simulink model "regbot_1mg_full"  (R2022b)
settings: Solver=ode15s  StartTime=0.0  StopTime=30  MaxStep=0.001  RelTol=1e-3  EnableMultiTasking=on
undefined symbols (not defined in the file or in its folder): alphaRT, alphaXV, BA, JA, K_PRT, K_PTV, K_PXV, Kemf, Kffwv, Kpwv, LA, mframe, mmotor, mtopextra, NG, pushDist, RA, startAngle, tau_dRT, tau_dTV, tau_dXV, tau_filter, tau_iRT, tau_iTV, tau_iXV, tau_post, tiwv, twvlp, WR, X, Y, Z
libraries: sm_lib x18, nesl_utility x9
settings Model: Creator=chr  LastModifiedBy=andre
settings SolverCC: AlgebraicLoopSolver=TrustRegion
settings DataIOCC: LimitDataPoints=on  SaveFormat=Array  ReturnWorkspaceOutputs=off
settings OptimizationCC: ExpressionDepthLimit=2147483647  LifeSpan=inf
settings DebuggingCC: UnderspecifiedInitializationDetection=Classic  MergeDetectMultiDrivingBlocksExec=none  SolverPrmCheckMsg=warning  UnconnectedInputMsg=warning  UnconnectedOutputMsg=warning  UnconnectedLineMsg=warning  StateNameClashWarn=warning  SFUnexpectedBacktrackingDiag=warning  SFNoUnconditionalDefaultTransitionDiag=warning  SFExecutionAtInitializationDiag=none  ArithmeticOperatorsInVariantConditions=warning
settings HardwareCC: ProdBitPerPointer=32  ProdBitPerSizeT=32  ProdBitPerPtrDiffT=32  ProdLargestAtomicFloat=None  ProdIntDivRoundTo=Undefined  ProdEndianess=Unspecified  ProdWordSize=32  ProdHWDeviceType=32-bit Generic
settings ModelReferenceCC: EnableRefExpFcnMdlSchedulingChecks=on  PropagateSignalLabelsOutOfModel=off
settings SFSimCC: SimUseLocalCustomCode=off  CustomCodeUndefinedFunction=UseInterfaceOnly
settings RTWCC: RTWUseLocalCustomCode=off  DLArmComputeVersion=19.05
settings CodeAppCC: StateflowObjectComments=on
settings GRTTargetCC: TargetLangStandard=C89/C90 (ANSI)
settings ConfigComp: CovMetricSettings=dw  CovSaveCumulativeToWorkspaceVar=on  CovSaveSingleToWorkspaceVar=on  CovExternalEMLEnable=off
settings SimscapeCC: SimscapeNormalizeSystem=off
settings ConfigurationSet: Description=SimMechanics 2G

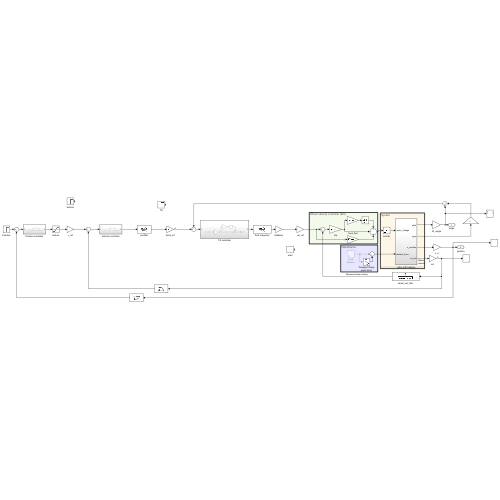
[thumbnail: Simulink's stored preview of the top-level diagram]
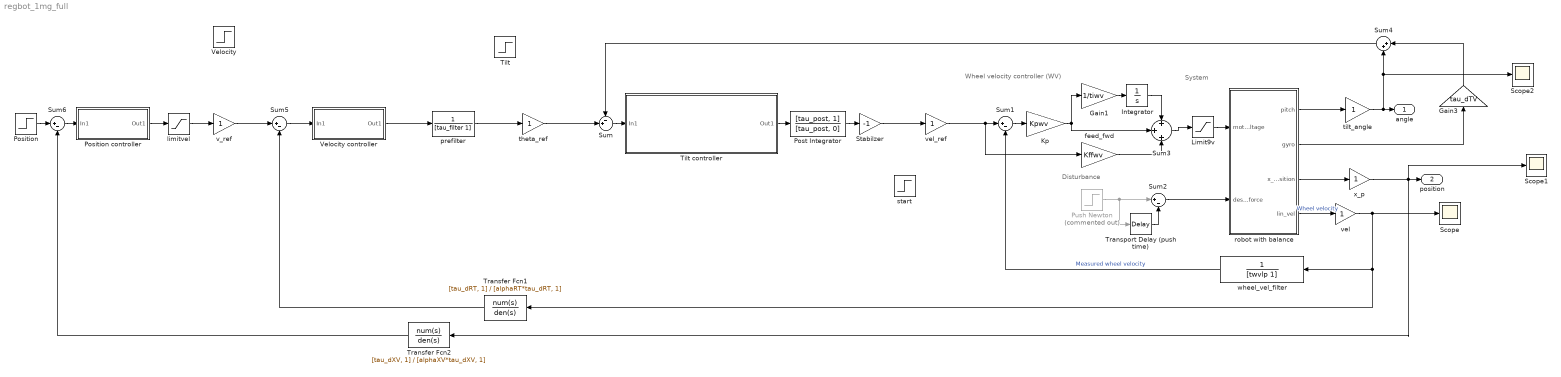
== system regbot_1mg_full ==
  note: System
  note: Disturbance
  note: Wheel velocity controller (WV)
  Gain1 : Gain  Gain=1/tiwv
  Gain3 : Gain  Gain=tau_dTV
  Integrator : Integrator  LimitOutput=on  UpperSaturationLimit=3  LowerSaturationLimit=-3
  Kp : Gain  Gain=Kpwv
  Limit9v : Saturate  UpperLimit=9  LowerLimit=-9
  Position : Step  Time=0  After=5  SampleTime=0
  Position controller : Subsystem
  Post Integrator : TransferFcn  Numerator=[tau_post, 1]  Denominator=[tau_post, 0]
  Push Newton : Step  Commented=on  After=2  SampleTime=0
  Scope : Scope
  Scope1 : Scope
  Scope2 : Scope
  Stabilzer : Gain  Gain=-1
  Sum : Sum  Inputs=-+|
  Sum{1..2,5..6} (4 alike) : Sum  Inputs=|+-
  Sum3 : Sum  Inputs=+|+|+
  Sum4 : Sum  Inputs=|++
  Tilt : Step  Time=0.2  After=3*pi/180  SampleTime=0
  Tilt controller : Subsystem
  Transfer Fcn1 : TransferFcn  Numerator=[tau_dRT, 1]  Denominator=[alphaRT*tau_dRT, 1]
  Transfer Fcn2 : TransferFcn  Numerator=[tau_dXV, 1]  Denominator=[alphaXV*tau_dXV, 1]
  Transport Delay (push time) : TransportDelay  DelayTime=0.1
  Velocity : Step  Time=0  After=0.8  SampleTime=0
  Velocity controller : Subsystem
  feed_fwd : Gain  Gain=Kffwv
  limitvel : Saturate  UpperLimit=1.2  LowerLimit=-1.2
  prefilter : TransferFcn  Denominator=[tau_filter 1]
  robot with balance : Subsystem
  start : Step  Time=0.2  After=1.1  SampleTime=0
  theta_ref : Gain
  tilt_angle : Gain
  v_ref : Gain
  vel : Gain
  vel_ref : Gain
  wheel_vel_filter : TransferFcn  Denominator=[twvlp 1]
  x_p : Gain
  angle : Outport  VectorParamsAs1DForOutWhenUnconnected=off
  position : Outport  Port=2  VectorParamsAs1DForOutWhenUnconnected=off
  wires:
  Push Newton/1 -> Transport Delay (push time)/1, Sum2/1
  Sum2/1 -> robot with balance/2(desturb_force)
  Transport Delay (push time)/1 -> Sum2/2
  Limit9v/1 -> robot with balance/1(motor_Voltage)
  Sum1/1 -> Kp/1
  Gain1/1 -> Integrator/1
  Integrator/1 -> Sum3/1
  Kp/1 -> Gain1/1, Sum3/2
  Sum3/1 -> Limit9v/1
  robot with balance/1(pitch) -> tilt_angle/1
  feed_fwd/1 -> Sum3/3
  wheel_vel_filter/1 -> Sum1/2  "Measured wheel velocity"
  vel_ref/1 -> feed_fwd/1, Sum1/1
  tilt_angle/1 -> Sum4/2, Scope2/1, angle/1
  Post Integrator/1 -> Stabilzer/1
  robot with balance/2(gyro) -> Gain3/1
  Sum4/1 -> Sum/1
  Sum/1 -> Tilt controller/1(In1)
  Gain3/1 -> Sum4/1
  Tilt controller/1(Out1) -> Post Integrator/1
  theta_ref/1 -> Sum/2
  Sum5/1 -> Velocity controller/1(In1)
  robot with balance/4(lin_vel) -> vel/1  "Wheel velocity"
  vel/1 -> Scope/1, Transfer Fcn1/1, wheel_vel_filter/1
  Velocity controller/1(Out1) -> prefilter/1
  Transfer Fcn1/1 -> Sum5/2
  robot with balance/3(x_position) -> x_p/1
  x_p/1 -> Scope1/1, position/1, Transfer Fcn2/1
  Position/1 -> Sum6/1
  Sum6/1 -> Position controller/1(In1)
  Transfer Fcn2/1 -> Sum6/2
  v_ref/1 -> Sum5/1
  Stabilzer/1 -> vel_ref/1
  prefilter/1 -> theta_ref/1
  Position controller/1(Out1) -> limitvel/1
  limitvel/1 -> v_ref/1

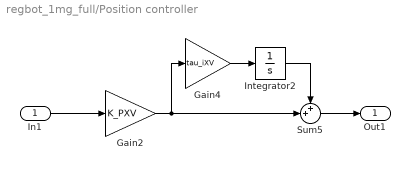
== system regbot_1mg_full/Position controller ==
  In1 : Inport
  Gain2 : Gain  Gain=K_PXV
  Gain4 : Gain  Gain=tau_iXV
  Integrator2 : Integrator  LimitOutput=on  UpperSaturationLimit=3  LowerSaturationLimit=-3
  Sum5 : Sum  Inputs=++|
  Out1 : Outport
  wires:
  Sum5/1 -> Out1/1
  In1/1 -> Gain2/1
  Gain4/1 -> Integrator2/1
  Gain2/1 -> Sum5/2, Gain4/1
  Integrator2/1 -> Sum5/1

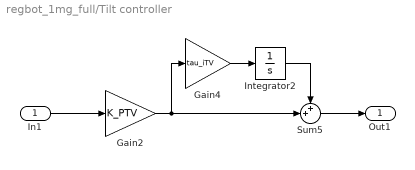
== system regbot_1mg_full/Tilt controller ==
  In1 : Inport
  Gain2 : Gain  Gain=K_PTV
  Gain4 : Gain  Gain=tau_iTV
  Integrator2 : Integrator  LimitOutput=on  UpperSaturationLimit=3  LowerSaturationLimit=-3
  Sum5 : Sum  Inputs=++|
  Out1 : Outport
  wires:
  Gain2/1 -> Gain4/1, Sum5/2
  Integrator2/1 -> Sum5/1
  Gain4/1 -> Integrator2/1
  Sum5/1 -> Out1/1
  In1/1 -> Gain2/1

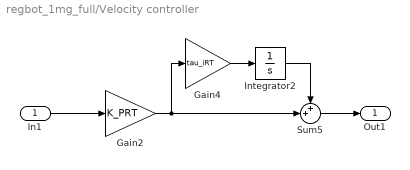
== system regbot_1mg_full/Velocity controller ==
  In1 : Inport
  Gain2 : Gain  Gain=K_PRT
  Gain4 : Gain  Gain=tau_iRT
  Integrator2 : Integrator  LimitOutput=on  UpperSaturationLimit=3  LowerSaturationLimit=-3
  Sum5 : Sum  Inputs=++|
  Out1 : Outport
  wires:
  Sum5/1 -> Out1/1
  In1/1 -> Gain2/1
  Gain4/1 -> Integrator2/1
  Gain2/1 -> Sum5/2, Gain4/1
  Integrator2/1 -> Sum5/1

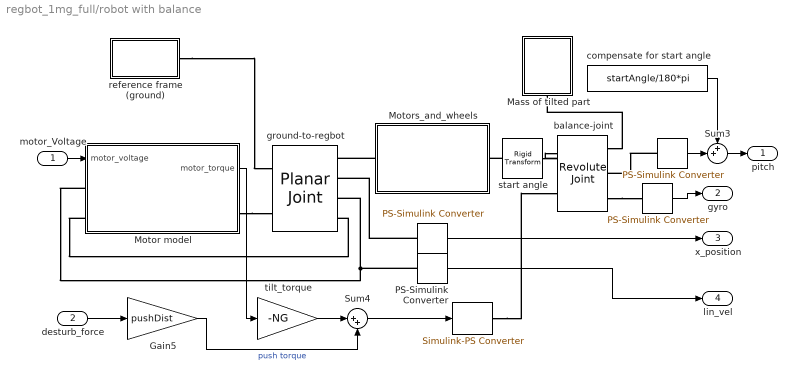
== system regbot_1mg_full/robot with balance ==
  motor_Voltage : Inport
  desturb_force : Inport  Port=2
  " " : nesl_utility/PS-Simulink Converter  PhysicalDomain=network_engine_domain  SubClassName=ps_output  LeftPortType=input  RightPortType=output  PseudoPeriodic=off  Frequencies=[]  VectorFormat=1-D array  Unit=1  AffineConversion=off
  "  " : nesl_utility/PS-Simulink Converter  PhysicalDomain=network_engine_domain  SubClassName=ps_output  LeftPortType=input  RightPortType=output  PseudoPeriodic=off  Frequencies=[]  VectorFormat=1-D array  Unit=1  AffineConversion=off
  "   " : nesl_utility/Simulink-PS Converter  PhysicalDomain=network_engine_domain  SubClassName=ps_input  LeftPortType=input  RightPortType=output  PseudoPeriodic=off  Frequencies=[]  NoiseDistribution=none  NoiseParameters=[]  Unit=1  AffineConversion=off  FilteringAndDerivatives=zero  SimscapeFilterOrder=1  InputFilterTimeConstant=.001  UdotUserProvided=[]
  "     " : nesl_utility/PS-Simulink Converter  PhysicalDomain=network_engine_domain  SubClassName=ps_output  LeftPortType=input  RightPortType=output  PseudoPeriodic=off  Frequencies=[]  VectorFormat=1-D array  Unit=1  AffineConversion=off
  Gain5 : Gain  Gain=pushDist
  Mass of tilted part : Subsystem
  Motor model : Subsystem
  Motors_and_wheels : Subsystem
  PS-Simulink Converter : nesl_utility/PS-Simulink Converter  PhysicalDomain=network_engine_domain  SubClassName=ps_output  LeftPortType=input  RightPortType=output  PseudoPeriodic=off  Frequencies=[]  VectorFormat=1-D array  Unit=1  AffineConversion=off
  Sum3 : Sum  Inputs=++|
  Sum4 : Sum  Inputs=|++
  balance-joint : sm_lib/Joints/Revolute Joint  JointMode=Normal  SenseConstraintForce=off  SenseConstraintForceX=off  SenseConstraintForceY=off  SenseConstraintForceZ=off  SenseConstraintTorque=off  SenseConstraintTorqueX=off  SenseConstraintTorqueY=off  SenseConstraintTorqueZ=off  SenseTotalForce=off  SenseTotalForceX=off  SenseTotalForceY=off  SenseTotalForceZ=off  SenseTotalTorque=off  SenseTotalTorqueX=off  SenseTotalTorqueY=off  SenseTotalTorqueZ=off  CompositeWrenchDir=FollowerOnBase  CompositeWrenchFrame=BaseFrame  EquilibriumPosition=0  EquilibriumPositionUnits=deg  SpringStiffness=0  SpringStiffnessUnits=N*m/deg  DampingCoefficient=0  DampingCoefficientUnits=N*m/(deg/s)  TorqueActuationMode=InputTorque  MotionActuationMode=ComputedMotion  SensePosition=on  SenseVelocity=on  SenseAcceleration=off  SenseTorqueForce=off  SenseLowerLimitTorqueForce=off  SenseUpperLimitTorqueForce=off  LowerLimitSpecify=off  LowerLimitBound=-90  LowerLimitBoundUnits=deg  LowerLimitStiffness=1e4  LowerLimitStiffnessUnits=N*m/deg  LowerLimitDamping=10  LowerLimitDampingUnits=N*m/(deg/s)  LowerLimitTransitionRegionWidth=0.1  LowerLimitTransitionRegionWidthUnits=deg  UpperLimitSpecify=off  UpperLimitBound=90  UpperLimitBoundUnits=deg  UpperLimitStiffness=1e4  UpperLimitStiffnessUnits=N*m/deg  UpperLimitDamping=10  UpperLimitDampingUnits=N*m/(deg/s)  UpperLimitTransitionRegionWidth=0.1  UpperLimitTransitionRegionWidthUnits=deg  PositionTargetSpecify=on  PositionTargetPriority=High  PositionTargetValue=0  PositionTargetValueUnits=deg  VelocityTargetSpecify=off  VelocityTargetPriority=High  VelocityTargetValue=0  VelocityTargetValueUnits=deg/s
  compensate for start angle : Constant  Value=startAngle/180*pi
  ground-to-regbot : sm_lib/Joints/Planar Joint  JointMode=Normal  SenseConstraintForce=off  SenseConstraintForceX=off  SenseConstraintForceY=off  SenseConstraintForceZ=off  SenseConstraintTorque=off  SenseConstraintTorqueX=off  SenseConstraintTorqueY=off  SenseConstraintTorqueZ=off  SenseTotalForce=off  SenseTotalForceX=off  SenseTotalForceY=off  SenseTotalForceZ=off  SenseTotalTorque=off  SenseTotalTorqueX=off  SenseTotalTorqueY=off  SenseTotalTorqueZ=off  CompositeWrenchDir=FollowerOnBase  CompositeWrenchFrame=BaseFrame  PxEquilibriumPosition=0  PxEquilibriumPositionUnits=m  PxSpringStiffness=0  PxSpringStiffnessUnits=N/m  PxDampingCoefficient=0.01  PxDampingCoefficientUnits=N/(m/s)  PxTorqueActuationMode=InputTorque  PxMotionActuationMode=ComputedMotion  PxSensePosition=on  PxSenseVelocity=on  PxSenseAcceleration=on  PxSenseTorqueForce=off  PxSenseLowerLimitTorqueForce=off  PxSenseUpperLimitTorqueForce=off  PxLowerLimitSpecify=off  PxLowerLimitBound=-1  PxLowerLimitBoundUnits=m  PxLowerLimitStiffness=1e6  PxLowerLimitStiffnessUnits=N/m  PxLowerLimitDamping=1e3  PxLowerLimitDampingUnits=N/(m/s)  PxLowerLimitTransitionRegionWidth=1e-4  PxLowerLimitTransitionRegionWidthUnits=m  PxUpperLimitSpecify=off  PxUpperLimitBound=1  PxUpperLimitBoundUnits=m  PxUpperLimitStiffness=1e6  PxUpperLimitStiffnessUnits=N/m  PxUpperLimitDamping=1e3  PxUpperLimitDampingUnits=N/(m/s)  PxUpperLimitTransitionRegionWidth=1e-4  PxUpperLimitTransitionRegionWidthUnits=m  PxPositionTargetSpecify=off  PxPositionTargetPriority=High  PxPositionTargetValue=0  PxPositionTargetValueUnits=m  PxVelocityTargetSpecify=off  PxVelocityTargetPriority=High  PxVelocityTargetValue=0  PxVelocityTargetValueUnits=m/s  PyEquilibriumPosition=0  PyEquilibriumPositionUnits=m  PySpringStiffness=1  PySpringStiffnessUnits=N/m  PyDampingCoefficient=1  PyDampingCoefficientUnits=N/(m/s)  PyTorqueActuationMode=NoTorque  PyMotionActuationMode=ComputedMotion  PySensePosition=off  PySenseVelocity=off  PySenseAcceleration=off  PySenseTorqueForce=off  PySenseLowerLimitTorqueForce=off  PySenseUpperLimitTorqueForce=off  PyLowerLimitSpecify=off  PyLowerLimitBound=-1  PyLowerLimitBoundUnits=m  PyLowerLimitStiffness=1e6  PyLowerLimitStiffnessUnits=N/m  PyLowerLimitDamping=1e3  PyLowerLimitDampingUnits=N/(m/s)  PyLowerLimitTransitionRegionWidth=1e-4  PyLowerLimitTransitionRegionWidthUnits=m  PyUpperLimitSpecify=off  PyUpperLimitBound=1  PyUpperLimitBoundUnits=m  PyUpperLimitStiffness=1e6  PyUpperLimitStiffnessUnits=N/m  PyUpperLimitDamping=1e3  PyUpperLimitDampingUnits=N/(m/s)  PyUpperLimitTransitionRegionWidth=1e-4  PyUpperLimitTransitionRegionWidthUnits=m  PyPositionTargetSpecify=off  PyPositionTargetPriority=High  PyPositionTargetValue=0  PyPositionTargetValueUnits=m  PyVelocityTargetSpecify=off  PyVelocityTargetPriority=High  PyVelocityTargetValue=0  PyVelocityTargetValueUnits=m/s  RzEquilibriumPosition=0  RzEquilibriumPositionUnits=deg  RzSpringStiffness=1  RzSpringStiffnessUnits=N*m/deg  RzDampingCoefficient=1  RzDampingCoefficientUnits=N*m/(deg/s)  RzTorqueActuationMode=NoTorque  RzMotionActuationMode=ComputedMotion  RzSensePosition=off  RzSenseVelocity=off  RzSenseAcceleration=off  RzSenseTorqueForce=off  RzSenseLowerLimitTorqueForce=off  RzSenseUpperLimitTorqueForce=off  RzLowerLimitSpecify=off  RzLowerLimitBound=-90  RzLowerLimitBoundUnits=deg  RzLowerLimitStiffness=1e4  RzLowerLimitStiffnessUnits=N*m/deg  RzLowerLimitDamping=10  RzLowerLimitDampingUnits=N*m/(deg/s)  RzLowerLimitTransitionRegionWidth=0.1  RzLowerLimitTransitionRegionWidthUnits=deg  RzUpperLimitSpecify=off  RzUpperLimitBound=90  RzUpperLimitBoundUnits=deg  RzUpperLimitStiffness=1e4  RzUpperLimitStiffnessUnits=N*m/deg  RzUpperLimitDamping=10  RzUpperLimitDampingUnits=N*m/(deg/s)  RzUpperLimitTransitionRegionWidth=0.1  RzUpperLimitTransitionRegionWidthUnits=deg  RzPositionTargetSpecify=off  RzPositionTargetPriority=High  RzPositionTargetValue=0  RzPositionTargetValueUnits=deg  RzVelocityTargetSpecify=off  RzVelocityTargetPriority=High  RzVelocityTargetValue=0  RzVelocityTargetValueUnits=deg/s
  reference frame (ground) : Subsystem
  start angle : sm_lib/Frames and Transforms/Rigid Transform  TranslationMethod=StandardAxis  TranslationStandardOffset=0.0  TranslationLengthUnit=m  TranslationStandardAxis=+Z  TranslationCartesianOffset=[0 0 0]  TranslationROffset=0  TranslationROffsetUnits=m  TranslationZOffset=0  TranslationZOffsetUnits=m  TranslationThetaOffset=0  TranslationThetaOffsetUnits=deg  RotationMethod=StandardAxis  RotationAngleUnits=deg  RotationStandardAxis=+Z  RotationAngle=startAngle  RotationArbitraryAxis=[0 0 1]  FollAlignAxisA=+X  BaseAlignAxisA=+X  FollAlignAxisB=+Z  BaseAlignAxisB=+Y  RotationSequenceAxes=FollowerAxes  RotationSequence=XYX  RotationSequenceAngles=[0 0 0]  RotationSequenceAnglesUnits=deg  RotationMatrix=[1 0 0; 0 1 0; 0 0 1]  Quaternion=[1 0 0 0]
  tilt_torque : Gain  Gain=-NG
  pitch : Outport  VectorParamsAs1DForOutWhenUnconnected=off
  gyro : Outport  Port=2  VectorParamsAs1DForOutWhenUnconnected=off
  x_position : Outport  Port=3  VectorParamsAs1DForOutWhenUnconnected=off
  lin_vel : Outport  Port=4  VectorParamsAs1DForOutWhenUnconnected=off
  wires:
  desturb_force/1 -> Gain5/1
  " "/1 -> gyro/1
  Sum4/1 -> "   "/1
  "  "/1 -> Sum3/2
  Sum3/1 -> pitch/1
  compensate for start angle/1 -> Sum3/1
  "     "/1 -> x_position/1
  PS-Simulink Converter/1 -> lin_vel/1
  motor_Voltage/1 -> Motor model/1(motor_voltage)
  Motor model/1(motor_torque) -> tilt_torque/1
  tilt_torque/1 -> Sum4/1
  Gain5/1 -> Sum4/2  "push torque"
  connections:
  "     "/LConn1 -- ground-to-regbot/RConn2
  balance-joint/RConn3 -- " "/LConn1
  "   "/RConn1 -- balance-joint/LConn2
  "  "/LConn1 -- balance-joint/RConn2
  start angle/RConn1 -- balance-joint/LConn1
  reference frame (ground)/RConn1 -- ground-to-regbot/LConn1
  PS-Simulink Converter/LConn1 -- Motor model/LConn1 -- ground-to-regbot/RConn3
  Motor model/RConn1 -- ground-to-regbot/LConn2
  Motor model/LConn2 -- ground-to-regbot/RConn4
  start angle/LConn1 -- Motors_and_wheels/RConn1
  Motors_and_wheels/LConn1 -- ground-to-regbot/RConn1
  balance-joint/RConn1 -- Mass of tilted part/LConn1

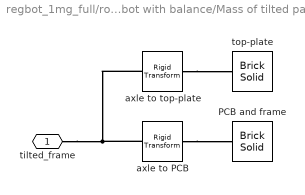
== system regbot_1mg_full/robot with balance/Mass of tilted part ==
  PCB and frame : sm_lib/Body Elements/Brick Solid  GraphicAmbientColor=[0.15 0.15 0.15 1.0]  BasedOnType=Mass  BrickDimensions=[0.005 0.1 0.1]  BrickDimensionUnits=m  CenterOfMass=[0 0 0]  CenterOfMassUnits=m  GraphicDiffuseColor=[0.2 0.7 0.2]  Density=1000  DensityUnits=kg/(m^3)  DoExposeReferenceFrame=on  GraphicEmissiveColor=[0.0 0.0 0.0 1.0]  ExportEntireGeometry=off  SerializedFrames=<Frames/>  MarkerShape=Sphere  MarkerSize=10  GraphicType=FromGeometry  InertiaType=CalculateFromGeometry  Mass=mframe  MassUnits=kg  MomentsOfInertia=[1 1 1]  MomentsOfInertiaUnits=kg*m^2  GraphicOpacity=1.0  ProductsOfInertia=[0 0 0]  ProductsOfInertiaUnits=kg*m^2  GraphicShininess=75  GraphicSpecularColor=[0.5 0.5 0.5 1.0]  GraphicVisPropType=SimpleVisualProperties
  axle to PCB : sm_lib/Frames and Transforms/Rigid Transform  TranslationMethod=StandardAxis  TranslationStandardOffset=0.055  TranslationLengthUnit=m  TranslationStandardAxis=-Y  TranslationCartesianOffset=[0 0 0]  TranslationROffset=0  TranslationROffsetUnits=m  TranslationZOffset=0  TranslationZOffsetUnits=m  TranslationThetaOffset=0  TranslationThetaOffsetUnits=deg  RotationMethod=StandardAxis  RotationAngleUnits=deg  RotationStandardAxis=+X  RotationAngle=90  RotationArbitraryAxis=[0 0 1]  FollAlignAxisA=+X  BaseAlignAxisA=+X  FollAlignAxisB=+Z  BaseAlignAxisB=+Y  RotationSequenceAxes=FollowerAxes  RotationSequence=XYX  RotationSequenceAngles=[0 0 0]  RotationSequenceAnglesUnits=deg  RotationMatrix=[1 0 0; 0 1 0; 0 0 1]  Quaternion=[1 0 0 0]
  axle to top-plate : sm_lib/Frames and Transforms/Rigid Transform  TranslationMethod=StandardAxis  TranslationStandardOffset=mpdist  TranslationLengthUnit=m  TranslationStandardAxis=-Y  TranslationCartesianOffset=[0 0.09 0]  TranslationROffset=0  TranslationROffsetUnits=m  TranslationZOffset=0  TranslationZOffsetUnits=m  TranslationThetaOffset=0  TranslationThetaOffsetUnits=deg  RotationMethod=StandardAxis  RotationAngleUnits=deg  RotationStandardAxis=+X  RotationAngle=90  RotationArbitraryAxis=[0 0 1]  FollAlignAxisA=+X  BaseAlignAxisA=+X  FollAlignAxisB=+Z  BaseAlignAxisB=+Y  RotationSequenceAxes=FollowerAxes  RotationSequence=XYX  RotationSequenceAngles=[0 0 0]  RotationSequenceAnglesUnits=deg  RotationMatrix=[1 0 0; 0 1 0; 0 0 1]  Quaternion=[1 0 0 0]
  top-plate : sm_lib/Body Elements/Brick Solid  GraphicAmbientColor=[0.15 0.15 0.15 1.0]  BasedOnType=Mass  BrickDimensions=[0.12 0.12 0.01]  BrickDimensionUnits=m  CenterOfMass=[0 0 0]  CenterOfMassUnits=m  GraphicDiffuseColor=[0.8 0.0 0.0]  Density=1000  DensityUnits=kg/(m^3)  DoExposeReferenceFrame=on  GraphicEmissiveColor=[0.0 0.0 0.0 1.0]  ExportEntireGeometry=off  SerializedFrames=<Frames/>  MarkerShape=Sphere  MarkerSize=10  GraphicType=FromGeometry  InertiaType=CalculateFromGeometry  Mass=mtopextra  MassUnits=kg  MomentsOfInertia=[1 1 1]  MomentsOfInertiaUnits=kg*m^2  GraphicOpacity=1.0  ProductsOfInertia=[0 0 0]  ProductsOfInertiaUnits=kg*m^2  GraphicShininess=75  GraphicSpecularColor=[0.5 0.5 0.5 1.0]  GraphicVisPropType=SimpleVisualProperties
  tilted_frame : PMIOPort  Side=Left
  connections:
  axle to PCB/RConn1 -- PCB and frame/RConn1
  axle to top-plate/LConn1 -- tilted_frame/RConn1 -- axle to PCB/LConn1
  axle to top-plate/RConn1 -- top-plate/RConn1

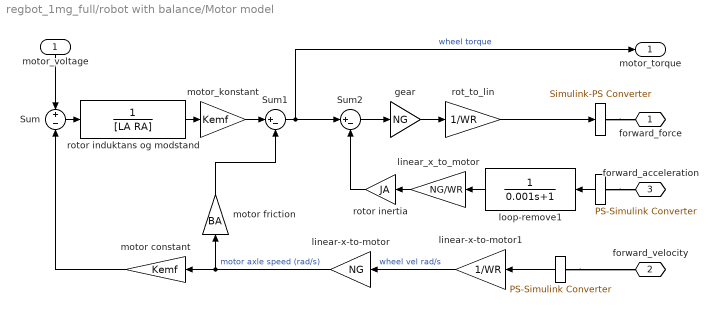
== system regbot_1mg_full/robot with balance/Motor model ==
  motor_voltage : Inport
  " " : nesl_utility/Simulink-PS Converter  PhysicalDomain=network_engine_domain  SubClassName=ps_input  LeftPortType=input  RightPortType=output  PseudoPeriodic=off  Frequencies=[]  NoiseDistribution=none  NoiseParameters=[]  Unit=1  AffineConversion=off  FilteringAndDerivatives=zero  SimscapeFilterOrder=1  InputFilterTimeConstant=.001  UdotUserProvided=[]
  "   " : nesl_utility/PS-Simulink Converter  PhysicalDomain=network_engine_domain  SubClassName=ps_output  LeftPortType=input  RightPortType=output  PseudoPeriodic=off  Frequencies=[]  VectorFormat=1-D array  Unit=1  AffineConversion=off
  "     " : nesl_utility/PS-Simulink Converter  PhysicalDomain=network_engine_domain  SubClassName=ps_output  LeftPortType=input  RightPortType=output  PseudoPeriodic=off  Frequencies=[]  VectorFormat=1-D array  Unit=1  AffineConversion=off
  Sum : Sum  Inputs=+|-
  Sum1 : Sum  Inputs=|+-
  Sum2 : Sum  Inputs=|+-
  gear : Gain  Gain=NG
  linear-x-to-motor : Gain  Gain=NG
  linear-x-to-motor1 : Gain  Gain=1/WR
  linear_x_to_motor : Gain  Gain=NG/WR
  loop-remove1 : TransferFcn  Denominator=[0.001 1]
  motor constant : Gain  Gain=Kemf
  motor friction : Gain  Gain=BA
  motor_konstant : Gain  Gain=Kemf
  rot_to_lin : Gain  Gain=1/WR
  rotor induktans og modstand : TransferFcn  Denominator=[LA RA]
  rotor inertia : Gain  Gain=JA
  forward_force : PMIOPort  Side=Right
  forward_velocity : PMIOPort  Port=2  Side=Left
  forward_acceleration : PMIOPort  Port=3  Side=Left
  motor_torque : Outport  VectorParamsAs1DForOutWhenUnconnected=off
  wires:
  Sum/1 -> rotor induktans og modstand/1
  rotor induktans og modstand/1 -> motor_konstant/1
  "     "/1 -> linear-x-to-motor1/1
  "   "/1 -> loop-remove1/1
  linear_x_to_motor/1 -> rotor inertia/1
  linear-x-to-motor/1 -> motor constant/1, motor friction/1  "motor axle speed (rad/s)"
  motor_konstant/1 -> Sum1/1
  Sum1/1 -> motor_torque/1, Sum2/1  "wheel torque"
  rotor inertia/1 -> Sum2/2
  motor constant/1 -> Sum/2
  rot_to_lin/1 -> " "/1
  motor friction/1 -> Sum1/2
  Sum2/1 -> gear/1
  loop-remove1/1 -> linear_x_to_motor/1
  motor_voltage/1 -> Sum/1
  gear/1 -> rot_to_lin/1
  linear-x-to-motor1/1 -> linear-x-to-motor/1  "wheel vel rad/s"
  connections:
  "     "/LConn1 -- forward_velocity/RConn1
  " "/RConn1 -- forward_force/RConn1
  "   "/LConn1 -- forward_acceleration/RConn1

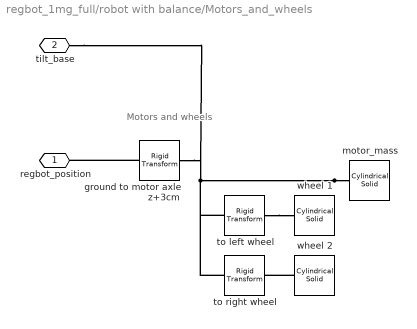
== system regbot_1mg_full/robot with balance/Motors_and_wheels ==
  note: Motors and wheels
  ground to motor axle z+3cm : sm_lib/Frames and Transforms/Rigid Transform  TranslationMethod=StandardAxis  TranslationStandardOffset=0.03  TranslationLengthUnit=m  TranslationStandardAxis=+Z  TranslationCartesianOffset=[0 0 0]  TranslationROffset=0  TranslationROffsetUnits=m  TranslationZOffset=0  TranslationZOffsetUnits=m  TranslationThetaOffset=0  TranslationThetaOffsetUnits=deg  RotationMethod=StandardAxis  RotationAngleUnits=deg  RotationStandardAxis=-X  RotationAngle=90  RotationArbitraryAxis=[0 0 1]  FollAlignAxisA=+X  BaseAlignAxisA=+X  FollAlignAxisB=+Z  BaseAlignAxisB=+Y  RotationSequenceAxes=FollowerAxes  RotationSequence=XYX  RotationSequenceAngles=[0 0 0]  RotationSequenceAnglesUnits=deg  RotationMatrix=[1 0 0; 0 1 0; 0 0 1]  Quaternion=[1 0 0 0]
  motor_mass : sm_lib/Body Elements/Cylindrical Solid  GraphicAmbientColor=[0.15 0.15 0.15 1.0]  BasedOnType=Mass  CenterOfMass=[0 0 0]  CenterOfMassUnits=m  GraphicDiffuseColor=[0.6 0.6 0.7]  CylinderLength=0.12  CylinderLengthUnits=m  CylinderRadius=0.012  CylinderRadiusUnits=m  Density=1000  DensityUnits=kg/(m^3)  DoExposeReferenceFrame=on  GraphicEmissiveColor=[0.0 0.0 0.0 1.0]  ExportEntireGeometry=off  SerializedFrames=<Frames/>  MarkerShape=Sphere  MarkerSize=10  GraphicType=FromGeometry  InertiaType=CalculateFromGeometry  Mass=mmotor  MassUnits=kg  MomentsOfInertia=[1 1 1]  MomentsOfInertiaUnits=kg*m^2  GraphicOpacity=1.0  ProductsOfInertia=[0 0 0]  ProductsOfInertiaUnits=kg*m^2  GraphicShininess=75  GraphicSpecularColor=[0.5 0.5 0.5 1.0]  GraphicVisPropType=SimpleVisualProperties
  to left wheel : sm_lib/Frames and Transforms/Rigid Transform  TranslationMethod=StandardAxis  TranslationStandardOffset=0.075  TranslationLengthUnit=m  TranslationStandardAxis=+Z  TranslationCartesianOffset=[0 0 0]  TranslationROffset=0  TranslationROffsetUnits=m  TranslationZOffset=0  TranslationZOffsetUnits=m  TranslationThetaOffset=0  TranslationThetaOffsetUnits=deg  RotationMethod=StandardAxis  RotationAngleUnits=deg  RotationStandardAxis=-X  RotationAngle=0  RotationArbitraryAxis=[0 0 1]  FollAlignAxisA=+X  BaseAlignAxisA=+X  FollAlignAxisB=+Z  BaseAlignAxisB=+Y  RotationSequenceAxes=FollowerAxes  RotationSequence=XYX  RotationSequenceAngles=[0 0 0]  RotationSequenceAnglesUnits=deg  RotationMatrix=[1 0 0; 0 1 0; 0 0 1]  Quaternion=[1 0 0 0]
  to right wheel : sm_lib/Frames and Transforms/Rigid Transform  TranslationMethod=StandardAxis  TranslationStandardOffset=0.075  TranslationLengthUnit=m  TranslationStandardAxis=-Z  TranslationCartesianOffset=[0 0 0]  TranslationROffset=0  TranslationROffsetUnits=m  TranslationZOffset=0  TranslationZOffsetUnits=m  TranslationThetaOffset=0  TranslationThetaOffsetUnits=deg  RotationMethod=StandardAxis  RotationAngleUnits=deg  RotationStandardAxis=-X  RotationAngle=0  RotationArbitraryAxis=[0 0 1]  FollAlignAxisA=+X  BaseAlignAxisA=+X  FollAlignAxisB=+Z  BaseAlignAxisB=+Y  RotationSequenceAxes=FollowerAxes  RotationSequence=XYX  RotationSequenceAngles=[0 0 0]  RotationSequenceAnglesUnits=deg  RotationMatrix=[1 0 0; 0 1 0; 0 0 1]  Quaternion=[1 0 0 0]
  wheel 1 : sm_lib/Body Elements/Cylindrical Solid  GraphicAmbientColor=[0.15 0.15 0.15 1.0]  BasedOnType=Mass  CenterOfMass=[0 0 0]  CenterOfMassUnits=m  GraphicDiffuseColor=[0.7 0.3 0.3]  CylinderLength=0.01  CylinderLengthUnits=m  CylinderRadius=0.03  CylinderRadiusUnits=m  Density=1000  DensityUnits=kg/(m^3)  DoExposeReferenceFrame=on  GraphicEmissiveColor=[0.0 0.0 0.0 1.0]  ExportEntireGeometry=off  SerializedFrames=<Frames/>  MarkerShape=Sphere  MarkerSize=10  GraphicType=FromGeometry  InertiaType=CalculateFromGeometry  Mass=0.01  MassUnits=kg  MomentsOfInertia=[1 1 1]  MomentsOfInertiaUnits=kg*m^2  GraphicOpacity=1.0  ProductsOfInertia=[0 0 0]  ProductsOfInertiaUnits=kg*m^2  GraphicShininess=75  GraphicSpecularColor=[0.5 0.5 0.5 1.0]  GraphicVisPropType=SimpleVisualProperties
  wheel 2 : sm_lib/Body Elements/Cylindrical Solid  GraphicAmbientColor=[0.15 0.15 0.15 1.0]  BasedOnType=Mass  CenterOfMass=[0 0 0]  CenterOfMassUnits=m  GraphicDiffuseColor=[0.7 0.3 0.3]  CylinderLength=0.01  CylinderLengthUnits=m  CylinderRadius=0.03  CylinderRadiusUnits=m  Density=1000  DensityUnits=kg/(m^3)  DoExposeReferenceFrame=on  GraphicEmissiveColor=[0.0 0.0 0.0 1.0]  ExportEntireGeometry=off  SerializedFrames=<Frames/>  MarkerShape=Sphere  MarkerSize=10  GraphicType=FromGeometry  InertiaType=CalculateFromGeometry  Mass=0.01  MassUnits=kg  MomentsOfInertia=[1 1 1]  MomentsOfInertiaUnits=kg*m^2  GraphicOpacity=1.0  ProductsOfInertia=[0 0 0]  ProductsOfInertiaUnits=kg*m^2  GraphicShininess=75  GraphicSpecularColor=[0.5 0.5 0.5 1.0]  GraphicVisPropType=SimpleVisualProperties
  regbot_position : PMIOPort  Side=Left
  tilt_base : PMIOPort  Port=2  Side=Right
  connections:
  motor_mass/RConn1 -- tilt_base/RConn1 -- ground to motor axle z+3cm/RConn1 -- to right wheel/LConn1 -- to left wheel/LConn1
  ground to motor axle z+3cm/LConn1 -- regbot_position/RConn1
  wheel 2/RConn1 -- to right wheel/RConn1
  to left wheel/RConn1 -- wheel 1/RConn1

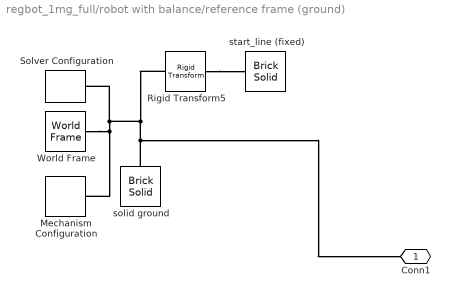
== system regbot_1mg_full/robot with balance/reference frame (ground) ==
  Mechanism Configuration : sm_lib/Utilities/Mechanism Configuration  UniformGravity=Constant  GravityVector=[0 0 -9.81]  GravityUnits=m/s^2  LinearizationDelta=0.001  JointModeTransitionNonlinearIterations=2
  Rigid Transform5 : sm_lib/Frames and Transforms/Rigid Transform  TranslationMethod=StandardAxis  TranslationStandardOffset=0.121  TranslationLengthUnit=m  TranslationStandardAxis=+Z  TranslationCartesianOffset=[0 0 0]  TranslationROffset=0  TranslationROffsetUnits=m  TranslationZOffset=0  TranslationZOffsetUnits=m  TranslationThetaOffset=0  TranslationThetaOffsetUnits=deg  RotationMethod=StandardAxis  RotationAngleUnits=deg  RotationStandardAxis=+Z  RotationAngle=0.  RotationArbitraryAxis=[0 0 1]  FollAlignAxisA=+X  BaseAlignAxisA=+X  FollAlignAxisB=+Z  BaseAlignAxisB=+Y  RotationSequenceAxes=FollowerAxes  RotationSequence=XYX  RotationSequenceAngles=[0 0 0]  RotationSequenceAnglesUnits=deg  RotationMatrix=[1 0 0; 0 1 0; 0 0 1]  Quaternion=[1 0 0 0]
  Solver Configuration : nesl_utility/Solver Configuration  PhysicalDomain=network_engine_domain  SubClassName=solver  LeftPortType=input  RightPortType=generic  Tones=[]  Harmonics=[]  SimulateNoise=off  Profile=off  UseLocalSampling=off  EnableSwitchedLinearOptims=on  FrequencyDomain=off  UseCCode=off  RelTol=0.001  AbsTol=1e-06  MinStep=1e-09  ToWorkspace=off  RevertToSquareIcSolve=off  NumHomotopyIterations=100  PhasorMode=off  PhasorModeNumHarmonics=1  ConsistencySolver=NEWTON_FTOL  IndexReductionMethod=DerivativeReplacement  DoDC=off  ResidualTolerance=1e-9  ConsistencyTolSource=GLOBAL  ConsistencyAbsTol=0.001  ConsistencyRelTol=0.001  ConsistencyTolFactor=0.001  UseLocalSolver=off  LocalSolverChoice=NE_BACKWARD_EULER_ADVANCER  ResolveIndetEquations=on  FunctionEvalNumThread=1  LocalSolverSampleTime=.001  DoFixedCost=off  MaxNonlinIter=3  MaxModeIter=2  ComputeImpulses=off  ImpulseIterations=2  LinearAlgebra=Sparse  LinearAlgebraNumThread=0  EquationFormulation=NE_TIME_EF  DelaysMemoryBudget=1024  AutomaticFiltering=on  FilteringTimeConstant=0.001  PartitionStorageMethod=AS_NEEDED  PartitionMemoryBudget=1024  PartitionMethod=FAST
  World Frame : sm_lib/Frames and Transforms/World Frame
  solid ground : sm_lib/Body Elements/Brick Solid  GraphicAmbientColor=[0.15 0.15 0.15 1.0]  BasedOnType=Density  BrickDimensions=[0.40 0.40 0.003]  BrickDimensionUnits=m  CenterOfMass=[0 0 0]  CenterOfMassUnits=m  GraphicDiffuseColor=[0.1 0.45 0]  Density=1000  DensityUnits=kg/(m^3)  DoExposeReferenceFrame=on  GraphicEmissiveColor=[0.0 0.0 0.0 1.0]  ExportEntireGeometry=off  SerializedFrames=<Frames/>  MarkerShape=Sphere  MarkerSize=10  GraphicType=FromGeometry  InertiaType=CalculateFromGeometry  Mass=1  MassUnits=kg  MomentsOfInertia=[1 1 1]  MomentsOfInertiaUnits=kg*m^2  GraphicOpacity=1.0  ProductsOfInertia=[0 0 0]  ProductsOfInertiaUnits=kg*m^2  GraphicShininess=75  GraphicSpecularColor=[0.5 0.5 0.5 1.0]  GraphicVisPropType=SimpleVisualProperties
  start_line (fixed) : sm_lib/Body Elements/Brick Solid  GraphicAmbientColor=[0.15 0.15 0.15 1.0]  BasedOnType=Mass  BrickDimensions=[0.001 0.04 0.25]  BrickDimensionUnits=m  CenterOfMass=[0 0 0]  CenterOfMassUnits=m  GraphicDiffuseColor=[0.4 0.4 0.7]  Density=1000  DensityUnits=kg/(m^3)  DoExposeReferenceFrame=on  GraphicEmissiveColor=[0.0 0.0 0.0 1.0]  ExportEntireGeometry=off  SerializedFrames=<Frames/>  MarkerShape=Sphere  MarkerSize=10  GraphicType=FromGeometry  InertiaType=CalculateFromGeometry  Mass=mtopextra  MassUnits=kg  MomentsOfInertia=[1 1 1]  MomentsOfInertiaUnits=kg*m^2  GraphicOpacity=1.0  ProductsOfInertia=[0 0 0]  ProductsOfInertiaUnits=kg*m^2  GraphicShininess=75  GraphicSpecularColor=[0.5 0.5 0.5 1.0]  GraphicVisPropType=SimpleVisualProperties
  Conn1 : PMIOPort  Side=Right
  connections:
  Solver Configuration/RConn1 -- World Frame/RConn1 -- Mechanism Configuration/RConn1 -- Rigid Transform5/LConn1 -- Conn1/RConn1 -- solid ground/RConn1
  Rigid Transform5/RConn1 -- start_line (fixed)/RConn1
